simulink model "youBot_Arm"  (R2024a)
settings: Solver=ode15s  StartTime=0.0  StopTime=20  MaxStep=1e-2  RelTol=1e-3  AbsTol=1e-4
model workspace: external: MATLAB File youBot_DataFile.m (data not in the file)
undefined symbols (not defined in the file): Extr_Data_LinkHoles, Qt, sigbuilder_block, smiData, tWP, X, Y, YBT_Par, Z
libraries: sm_lib x193, nesl_utility x130, fl_lib x53, simulink x13, Parts_Lib x10, MyMath_lib x8, Motor_Lib x5, Contact_Forces_Lib x4, ee_lib x2, sdl_lib x2
(part 7 of 8)

== system youBot_Arm/Arm/Environment/Gripper Force/Damper/Gripper Force ==
  Force : Subsystem  mask(Controlled 6-DOF Damping Force){b=contact_b, lpfilt_const_force=lpf_const_gripper_force}
      mask prompts: b "Damping Coefficient"; lpfilt_const_force "Low Pass Filter Constant"
      mask help: Models a controlled 6-DOF damping force. If the distance between two frames is within a certain range (px, py, pz), the damping force is active.
  Measure Apply 6-DOF : sm_lib/Joints/6-DOF Joint  JointMode=Normal  CompositeWrenchDir=FollowerOnBase  CompositeWrenchFrame=BaseFrame  SenseConstraintForce=off  SenseConstraintTorque=off  SenseTotalForce=off  SenseTotalTorque=off  PxPositionTargetSpecify=off  PxPositionTargetPriority=High  PxPositionTargetValue=0  PxPositionTargetValueUnits=m  PxVelocityTargetSpecify=off  PxVelocityTargetPriority=High  PxVelocityTargetValue=0  PxVelocityTargetValueUnits=m/s  PxEquilibriumPosition=0  PxEquilibriumPositionUnits=m  PxSpringStiffness=0  PxSpringStiffnessUnits=N/m  PxDampingCoefficient=0  PxDampingCoefficientUnits=N/(m/s)  PxLowerLimitSpecify=off  PxLowerLimitBound=-1  PxLowerLimitBoundUnits=m  PxLowerLimitStiffness=1e6  PxLowerLimitStiffnessUnits=N/m  PxLowerLimitDamping=1e3  PxLowerLimitDampingUnits=N/(m/s)  PxLowerLimitTransitionRegionWidth=1e-4  PxLowerLimitTransitionRegionWidthUnits=m  PxUpperLimitSpecify=off  PxUpperLimitBound=1  PxUpperLimitBoundUnits=m  PxUpperLimitStiffness=1e6  PxUpperLimitStiffnessUnits=N/m  PxUpperLimitDamping=1e3  PxUpperLimitDampingUnits=N/(m/s)  PxUpperLimitTransitionRegionWidth=1e-4  PxUpperLimitTransitionRegionWidthUnits=m  PxTorqueActuationMode=InputTorque  PxMotionActuationMode=ComputedMotion  PxSensePosition=on  PxSenseVelocity=on  PxSenseAcceleration=off  PxSenseTorqueForce=off  PxSenseLowerLimitTorqueForce=off  PxSenseUpperLimitTorqueForce=off  PyPositionTargetSpecify=off  PyPositionTargetPriority=High  PyPositionTargetValue=40e-2  PyPositionTargetValueUnits=m  PyVelocityTargetSpecify=off  PyVelocityTargetPriority=High  PyVelocityTargetValue=0  PyVelocityTargetValueUnits=m/s  PyEquilibriumPosition=0  PyEquilibriumPositionUnits=m  PySpringStiffness=0  PySpringStiffnessUnits=N/m  PyDampingCoefficient=0  PyDampingCoefficientUnits=N/(m/s)  PyLowerLimitSpecify=off  PyLowerLimitBound=-1  PyLowerLimitBoundUnits=m  PyLowerLimitStiffness=1e6  PyLowerLimitStiffnessUnits=N/m  PyLowerLimitDamping=1e3  PyLowerLimitDampingUnits=N/(m/s)  PyLowerLimitTransitionRegionWidth=1e-4  PyLowerLimitTransitionRegionWidthUnits=m  PyUpperLimitSpecify=off  PyUpperLimitBound=1  PyUpperLimitBoundUnits=m  PyUpperLimitStiffness=1e6  PyUpperLimitStiffnessUnits=N/m  PyUpperLimitDamping=1e3  PyUpperLimitDampingUnits=N/(m/s)  PyUpperLimitTransitionRegionWidth=1e-4  PyUpperLimitTransitionRegionWidthUnits=m  PyTorqueActuationMode=InputTorque  PyMotionActuationMode=ComputedMotion  PySensePosition=on  PySenseVelocity=on  PySenseAcceleration=off  PySenseTorqueForce=off  PySenseLowerLimitTorqueForce=off  PySenseUpperLimitTorqueForce=off  PzPositionTargetSpecify=off  PzPositionTargetPriority=High  PzPositionTargetValue=(YBT_Par.Floor.d+YBT_Par.Cube.d)/2+0.1  PzPositionTargetValueUnits=m  PzVelocityTargetSpecify=off  PzVelocityTargetPriority=High  PzVelocityTargetValue=0  PzVelocityTargetValueUnits=m/s  PzEquilibriumPosition=0  PzEquilibriumPositionUnits=m  PzSpringStiffness=0  PzSpringStiffnessUnits=N/m  PzDampingCoefficient=0  PzDampingCoefficientUnits=N/(m/s)  PzLowerLimitSpecify=off  PzLowerLimitBound=-1  PzLowerLimitBoundUnits=m  PzLowerLimitStiffness=1e6  PzLowerLimitStiffnessUnits=N/m  PzLowerLimitDamping=1e3  PzLowerLimitDampingUnits=N/(m/s)  PzLowerLimitTransitionRegionWidth=1e-4  PzLowerLimitTransitionRegionWidthUnits=m  PzUpperLimitSpecify=off  PzUpperLimitBound=1  PzUpperLimitBoundUnits=m  PzUpperLimitStiffness=1e6  PzUpperLimitStiffnessUnits=N/m  PzUpperLimitDamping=1e3  PzUpperLimitDampingUnits=N/(m/s)  PzUpperLimitTransitionRegionWidth=1e-4  PzUpperLimitTransitionRegionWidthUnits=m  PzTorqueActuationMode=InputTorque  PzMotionActuationMode=ComputedMotion  PzSensePosition=on  PzSenseVelocity=on  PzSenseAcceleration=off  PzSenseTorqueForce=off  PzSenseLowerLimitTorqueForce=off  PzSenseUpperLimitTorqueForce=off  SphPositionTargetSpecify=off  SphPositionTargetPriority=High  SphPositionTargetRotationMethod=None  SphPositionTargetFollAlignAxisA=+X  SphPositionTargetBaseAlignAxisA=+Y  SphPositionTargetFollAlignAxisB=+Y  SphPositionTargetBaseAlignAxisB=+Z  SphPositionTargetRotationStandardAxis=+Z  SphPositionTargetRotationAngle=0.0  SphPositionTargetRotationAngleUnits=deg  SphPositionTargetRotationArbitraryAxis=[0 0 1]  SphPositionTargetRotationSequenceAxes=FollowerAxes  SphPositionTargetRotationSequence=XYX  SphPositionTargetRotationSequenceAngles=[0 0 0]  SphPositionTargetRotationSequenceAnglesUnits=deg  SphPositionTargetRotationMatrix=[1 0 0; 0 1 0; 0 0 1]  SphPositionTargetQuaternion=[1 0 0 0]  SphVelocityTargetSpecify=off  SphVelocityTargetPriority=High  SphVelocityTargetValue=[0 0 0]  SphVelocityTargetValueUnits=deg/s  SphVelocityTargetInFollowerFrame=on  SphEqPosRotationMethod=None  SphEqPosFollAlignAxisA=+X  SphEqPosBaseAlignAxisA=+Y  SphEqPosFollAlignAxisB=+Y  SphEqPosBaseAlignAxisB=+Z  SphEqPosRotationStandardAxis=+Z  SphEqPosRotationAngle=0.0  SphEqPosRotationAngleUnits=deg  SphEqPosRotationArbitraryAxis=[0 0 1]  SphEqPosRotationSequenceAxes=FollowerAxes  SphEqPosRotationSequence=XYX  SphEqPosRotationSequenceAngles=[0 0 0]  SphEqPosRotationSequenceAnglesUnits=deg  SphEqPosRotationMatrix=[1 0 0; 0 1 0; 0 0 1]  SphEqPosQuaternion=[1 0 0 0]  SphSpringStiffness=0  SphSpringStiffnessUnits=N*m/deg  SphDampingCoefficient=0  SphDampingCoefficientUnits=N*m/(deg/s)  SphLowerLimitSpecify=off  SphLowerLimitBound=15  SphLowerLimitBoundUnits=deg  SphLowerLimitStiffness=1e4  SphLowerLimitStiffnessUnits=N*m/deg  SphLowerLimitDamping=10  SphLowerLimitDampingUnits=N*m/(deg/s)  SphLowerLimitTransitionRegionWidth=0.1  SphLowerLimitTransitionRegionWidthUnits=deg  SphUpperLimitSpecify=off  SphUpperLimitBound=45  SphUpperLimitBoundUnits=deg  SphUpperLimitStiffness=1e4  SphUpperLimitStiffnessUnits=N*m/deg  SphUpperLimitDamping=10  SphUpperLimitDampingUnits=N*m/(deg/s)  SphUpperLimitTransitionRegionWidth=0.1  SphUpperLimitTransitionRegionWidthUnits=deg  SphTorqueActuationMode=InputTorque  SphActuateTorqueX=on  SphActuateTorqueY=on  SphActuateTorqueZ=on  SphActuateTorque=off  SphActuationFrame=BaseFrame  SphSensePosition=off  SphSenseVelocityX=on  SphSenseVelocityY=on  SphSenseVelocityZ=on  SphSenseVelocity=off  SphSenseAccelerationX=off  SphSenseAccelerationY=off  SphSenseAccelerationZ=off  SphSenseAcceleration=off  SphSenseLowerLimitTorqueMag=off  SphSenseUpperLimitTorqueMag=off  SphSensingFrame=BaseFrame
  Relative vz : Subsystem  Variant=on  VariantControlMode=label  LabelModeActiveChoice=Housing
      settings: AttributesFormatString=%<ActiveVariant>
  b : PMIOPort  Side=Right
  E : PMIOPort  Port=2  Side=Right
  a : PMIOPort  Port=3  Side=Right
  Box : PMIOPort  Port=4  Side=Left
  connections:
  Force/LConn9 -- Measure Apply 6-DOF/RConn2
  Force/LConn7 -- Measure Apply 6-DOF/RConn4
  Force/LConn5 -- Measure Apply 6-DOF/RConn6
  Force/RConn4 -- Measure Apply 6-DOF/LConn4
  Force/LConn2 -- Measure Apply 6-DOF/RConn9
  Measure Apply 6-DOF/RConn8 -- Force/LConn3
  Force/RConn2 -- Measure Apply 6-DOF/LConn6
  Force/RConn3 -- Measure Apply 6-DOF/LConn5
  Force/RConn6 -- Measure Apply 6-DOF/LConn2
  Measure Apply 6-DOF/LConn3 -- Force/RConn5
  Measure Apply 6-DOF/RConn3 -- Force/LConn8
  Force/LConn6 -- Measure Apply 6-DOF/RConn5
  Force/LConn1 -- Measure Apply 6-DOF/RConn10
  Measure Apply 6-DOF/LConn1 -- a/RConn1
  Measure Apply 6-DOF/RConn1 -- Relative vz/LConn2 -- Box/RConn1
  Measure Apply 6-DOF/LConn7 -- Force/RConn1
  Relative vz/LConn3 -- b/RConn1
  Relative vz/LConn4 -- E/RConn1
  Relative vz/LConn1 -- Measure Apply 6-DOF/RConn7
  Relative vz/RConn1 -- Force/LConn4

== system youBot_Arm/Arm/Environment/Gripper Force/Payload/Marks ==
  Front Rear : sm_lib/Body Elements/Extruded Solid  ExtrusionType=General  PolygonNumSides=3  PolygonOuterRadius=1  PolygonOuterRadiusUnits=m  ExportEntireGeometry=off  ExtrusionCrossSection=YBT_Par.Cube.mark.extrusion  ExtrusionCrossSectionUnits=m  ExportConvexHullGeometry=off  ExtrusionLength=YBT_Par.Cube.d*1.001  ExtrusionLengthUnits=m  InertiaType=PointMass  BasedOnType=Density  Density=1000  DensityUnits=kg/m^3  Mass=0  MassUnits=kg  CenterOfMass=[0 0 0]  CenterOfMassUnits=m  MomentsOfInertia=[1 1 1]  MomentsOfInertiaUnits=kg*m^2  ProductsOfInertia=[1 1 1]  ProductsOfInertiaUnits=kg*m^2  GraphicType=FromGeometry  MarkerShape=Sphere  MarkerSize=10  GraphicVisPropType=SimpleVisualProperties  GraphicDiffuseColor=YBT_Par.Cube.mark.color  GraphicOpacity=1  GraphicSpecularColor=[0.5 0.5 0.5 1.0]  GraphicAmbientColor=[0.15 0.15 0.15 1.0]  GraphicEmissiveColor=[0.0 0.0 0.0 1.0]  GraphicShininess=75  DoExposeReferenceFrame=on  SerializedFrames=<Frames/>
  Left Right : sm_lib/Body Elements/Extruded Solid  ExtrusionType=General  PolygonNumSides=3  PolygonOuterRadius=1  PolygonOuterRadiusUnits=m  ExportEntireGeometry=off  ExtrusionCrossSection=YBT_Par.Cube.mark.extrusion  ExtrusionCrossSectionUnits=m  ExportConvexHullGeometry=off  ExtrusionLength=YBT_Par.Cube.d*1.001  ExtrusionLengthUnits=m  InertiaType=PointMass  BasedOnType=Density  Density=1000  DensityUnits=kg/m^3  Mass=0  MassUnits=kg  CenterOfMass=[0 0 0]  CenterOfMassUnits=m  MomentsOfInertia=[1 1 1]  MomentsOfInertiaUnits=kg*m^2  ProductsOfInertia=[1 1 1]  ProductsOfInertiaUnits=kg*m^2  GraphicType=FromGeometry  MarkerShape=Sphere  MarkerSize=10  GraphicVisPropType=SimpleVisualProperties  GraphicDiffuseColor=YBT_Par.Cube.mark.color  GraphicOpacity=1  GraphicSpecularColor=[0.5 0.5 0.5 1.0]  GraphicAmbientColor=[0.15 0.15 0.15 1.0]  GraphicEmissiveColor=[0.0 0.0 0.0 1.0]  GraphicShininess=75  DoExposeReferenceFrame=on  SerializedFrames=<Frames/>
  Transform Mark Front Rear : sm_lib/Frames and Transforms/Rigid Transform  RotationMethod=StandardAxis  FollAlignAxisA=+X  BaseAlignAxisA=+Y  FollAlignAxisB=+Y  BaseAlignAxisB=+Z  RotationStandardAxis=+X  RotationAngle=90  RotationAngleUnits=deg  RotationArbitraryAxis=[0 0 1]  RotationSequenceAxes=FollowerAxes  RotationSequence=XYX  RotationSequenceAngles=[0 0 0]  RotationSequenceAnglesUnits=deg  RotationMatrix=[1 0 0; 0 1 0; 0 0 1]  Quaternion=[1 0 0 0]  TranslationMethod=None  TranslationCartesianOffset=[0 0 0]  TranslationCartesianOffsetUnits=m  TranslationStandardAxis=+Z  TranslationStandardOffset=0  TranslationStandardOffsetUnits=m  TranslationROffset=0  TranslationROffsetUnits=m  TranslationThetaOffset=0  TranslationThetaOffsetUnits=deg  TranslationZOffset=0  TranslationZOffsetUnits=m
  Transform Mark Left Right : sm_lib/Frames and Transforms/Rigid Transform  RotationMethod=StandardAxis  FollAlignAxisA=+X  BaseAlignAxisA=+Y  FollAlignAxisB=+Y  BaseAlignAxisB=+Z  RotationStandardAxis=+Y  RotationAngle=90  RotationAngleUnits=deg  RotationArbitraryAxis=[0 0 1]  RotationSequenceAxes=FollowerAxes  RotationSequence=XYX  RotationSequenceAngles=[0 0 0]  RotationSequenceAnglesUnits=deg  RotationMatrix=[1 0 0; 0 1 0; 0 0 1]  Quaternion=[1 0 0 0]  TranslationMethod=None  TranslationCartesianOffset=[0 0 0]  TranslationCartesianOffsetUnits=m  TranslationStandardAxis=+Z  TranslationStandardOffset=0  TranslationStandardOffsetUnits=m  TranslationROffset=0  TranslationROffsetUnits=m  TranslationThetaOffset=0  TranslationThetaOffsetUnits=deg  TranslationZOffset=0  TranslationZOffsetUnits=m
  R : PMIOPort  Side=Left
  connections:
  Left Right/RConn1 -- Transform Mark Left Right/RConn1
  Transform Mark Front Rear/RConn1 -- Front Rear/RConn1 -- Transform Mark Left Right/LConn1
  Transform Mark Front Rear/LConn1 -- R/RConn1

== system youBot_Arm/Arm/Environment/Gripper Force/Penalty/Sc2 ==
  In1 : Inport
  Bus Selector1 : BusSelector  OutputSignals=fz1.Normal Force,fz1.Friction Force,fz2.Normal Force,fz2.Friction Force,fz3.Normal Force,fz3.Friction Force,fz4.Normal Force,fz4.Friction Force
  Scope1 : Scope  NumInputPorts=8
  wires:
  Bus Selector1/8 -> Scope1/8  "<Friction Force>"
  Bus Selector1/7 -> Scope1/7  "<Normal Force>"
  Bus Selector1/5 -> Scope1/5  "<Normal Force>"
  In1/1 -> Bus Selector1/1
  Bus Selector1/6 -> Scope1/6  "<Friction Force>"
  Bus Selector1/2 -> Scope1/2  "<Friction Force>"
  Bus Selector1/4 -> Scope1/4  "<Friction Force>"
  Bus Selector1/3 -> Scope1/3  "<Normal Force>"
  Bus Selector1/1 -> Scope1/1  "<Normal Force>"

== system youBot_Arm/Arm/Environment/Load/Box/Camera Frames ==
  Box Left : sm_lib/Frames and Transforms/Rigid Transform  RotationMethod=None  FollAlignAxisA=+X  BaseAlignAxisA=+Y  FollAlignAxisB=+Y  BaseAlignAxisB=+Z  RotationStandardAxis=+Z  RotationAngle=0.0  RotationAngleUnits=deg  RotationArbitraryAxis=[0 0 1]  RotationSequenceAxes=FollowerAxes  RotationSequence=XYX  RotationSequenceAngles=[0 0 0]  RotationSequenceAnglesUnits=deg  RotationMatrix=[1 0 0; 0 1 0; 0 0 1]  Quaternion=[1 0 0 0]  TranslationMethod=StandardAxis  TranslationCartesianOffset=[0 0 0]  TranslationCartesianOffsetUnits=m  TranslationStandardAxis=+X  TranslationStandardOffset=YBT_Par.Cube.d/2+2e-1  TranslationStandardOffsetUnits=m  TranslationROffset=0  TranslationROffsetUnits=m  TranslationThetaOffset=0  TranslationThetaOffsetUnits=deg  TranslationZOffset=0  TranslationZOffsetUnits=m
  Box Rear : sm_lib/Frames and Transforms/Rigid Transform  RotationMethod=None  FollAlignAxisA=+X  BaseAlignAxisA=+Y  FollAlignAxisB=+Y  BaseAlignAxisB=+Z  RotationStandardAxis=+Z  RotationAngle=0.0  RotationAngleUnits=deg  RotationArbitraryAxis=[0 0 1]  RotationSequenceAxes=FollowerAxes  RotationSequence=XYX  RotationSequenceAngles=[0 0 0]  RotationSequenceAnglesUnits=deg  RotationMatrix=[1 0 0; 0 1 0; 0 0 1]  Quaternion=[1 0 0 0]  TranslationMethod=StandardAxis  TranslationCartesianOffset=[0 0 0]  TranslationCartesianOffsetUnits=m  TranslationStandardAxis=+Y  TranslationStandardOffset=YBT_Par.Cube.d/2+2e-1  TranslationStandardOffsetUnits=m  TranslationROffset=0  TranslationROffsetUnits=m  TranslationThetaOffset=0  TranslationThetaOffsetUnits=deg  TranslationZOffset=0  TranslationZOffsetUnits=m
  Box Right : sm_lib/Frames and Transforms/Rigid Transform  RotationMethod=None  FollAlignAxisA=+X  BaseAlignAxisA=+Y  FollAlignAxisB=+Y  BaseAlignAxisB=+Z  RotationStandardAxis=+Z  RotationAngle=0.0  RotationAngleUnits=deg  RotationArbitraryAxis=[0 0 1]  RotationSequenceAxes=FollowerAxes  RotationSequence=XYX  RotationSequenceAngles=[0 0 0]  RotationSequenceAnglesUnits=deg  RotationMatrix=[1 0 0; 0 1 0; 0 0 1]  Quaternion=[1 0 0 0]  TranslationMethod=StandardAxis  TranslationCartesianOffset=[0 0 0]  TranslationCartesianOffsetUnits=m  TranslationStandardAxis=-X  TranslationStandardOffset=YBT_Par.Cube.d/2+2e-1  TranslationStandardOffsetUnits=m  TranslationROffset=0  TranslationROffsetUnits=m  TranslationThetaOffset=0  TranslationThetaOffsetUnits=deg  TranslationZOffset=0  TranslationZOffsetUnits=m
  B : PMIOPort  Side=Left
  connections:
  Box Rear/LConn1 -- Box Left/LConn1 -- Box Right/LConn1 -- B/RConn1

== system youBot_Arm/Arm/Environment/Load/Box/Marks ==
  Front Rear : sm_lib/Body Elements/Extruded Solid  ExtrusionType=General  PolygonNumSides=3  PolygonOuterRadius=1  PolygonOuterRadiusUnits=m  ExportEntireGeometry=off  ExtrusionCrossSection=YBT_Par.Cube.mark.extrusion  ExtrusionCrossSectionUnits=m  ExportConvexHullGeometry=off  ExtrusionLength=YBT_Par.Cube.d*1.001  ExtrusionLengthUnits=m  InertiaType=PointMass  BasedOnType=Density  Density=1000  DensityUnits=kg/m^3  Mass=0  MassUnits=kg  CenterOfMass=[0 0 0]  CenterOfMassUnits=m  MomentsOfInertia=[1 1 1]  MomentsOfInertiaUnits=kg*m^2  ProductsOfInertia=[1 1 1]  ProductsOfInertiaUnits=kg*m^2  GraphicType=FromGeometry  MarkerShape=Sphere  MarkerSize=10  GraphicVisPropType=SimpleVisualProperties  GraphicDiffuseColor=YBT_Par.Cube.mark.color  GraphicOpacity=1.0  GraphicSpecularColor=[0.5 0.5 0.5 1.0]  GraphicAmbientColor=[0.15 0.15 0.15 1.0]  GraphicEmissiveColor=[0.0 0.0 0.0 1.0]  GraphicShininess=75  DoExposeReferenceFrame=on  SerializedFrames=<Frames/>
  Left Right : sm_lib/Body Elements/Extruded Solid  ExtrusionType=General  PolygonNumSides=3  PolygonOuterRadius=1  PolygonOuterRadiusUnits=m  ExportEntireGeometry=off  ExtrusionCrossSection=YBT_Par.Cube.mark.extrusion  ExtrusionCrossSectionUnits=m  ExportConvexHullGeometry=off  ExtrusionLength=YBT_Par.Cube.d*1.001  ExtrusionLengthUnits=m  InertiaType=PointMass  BasedOnType=Density  Density=1000  DensityUnits=kg/m^3  Mass=0  MassUnits=kg  CenterOfMass=[0 0 0]  CenterOfMassUnits=m  MomentsOfInertia=[1 1 1]  MomentsOfInertiaUnits=kg*m^2  ProductsOfInertia=[1 1 1]  ProductsOfInertiaUnits=kg*m^2  GraphicType=FromGeometry  MarkerShape=Sphere  MarkerSize=10  GraphicVisPropType=SimpleVisualProperties  GraphicDiffuseColor=YBT_Par.Cube.mark.color  GraphicOpacity=1.0  GraphicSpecularColor=[0.5 0.5 0.5 1.0]  GraphicAmbientColor=[0.15 0.15 0.15 1.0]  GraphicEmissiveColor=[0.0 0.0 0.0 1.0]  GraphicShininess=75  DoExposeReferenceFrame=on  SerializedFrames=<Frames/>
  Transform Mark Front Rear : sm_lib/Frames and Transforms/Rigid Transform  RotationMethod=StandardAxis  FollAlignAxisA=+X  BaseAlignAxisA=+Y  FollAlignAxisB=+Y  BaseAlignAxisB=+Z  RotationStandardAxis=+X  RotationAngle=90  RotationAngleUnits=deg  RotationArbitraryAxis=[0 0 1]  RotationSequenceAxes=FollowerAxes  RotationSequence=XYX  RotationSequenceAngles=[0 0 0]  RotationSequenceAnglesUnits=deg  RotationMatrix=[1 0 0; 0 1 0; 0 0 1]  Quaternion=[1 0 0 0]  TranslationMethod=None  TranslationCartesianOffset=[0 0 0]  TranslationCartesianOffsetUnits=m  TranslationStandardAxis=+Z  TranslationStandardOffset=0  TranslationStandardOffsetUnits=m  TranslationROffset=0  TranslationROffsetUnits=m  TranslationThetaOffset=0  TranslationThetaOffsetUnits=deg  TranslationZOffset=0  TranslationZOffsetUnits=m
  Transform Mark Left Right : sm_lib/Frames and Transforms/Rigid Transform  RotationMethod=StandardAxis  FollAlignAxisA=+X  BaseAlignAxisA=+Y  FollAlignAxisB=+Y  BaseAlignAxisB=+Z  RotationStandardAxis=+Y  RotationAngle=90  RotationAngleUnits=deg  RotationArbitraryAxis=[0 0 1]  RotationSequenceAxes=FollowerAxes  RotationSequence=XYX  RotationSequenceAngles=[0 0 0]  RotationSequenceAnglesUnits=deg  RotationMatrix=[1 0 0; 0 1 0; 0 0 1]  Quaternion=[1 0 0 0]  TranslationMethod=None  TranslationCartesianOffset=[0 0 0]  TranslationCartesianOffsetUnits=m  TranslationStandardAxis=+Z  TranslationStandardOffset=0  TranslationStandardOffsetUnits=m  TranslationROffset=0  TranslationROffsetUnits=m  TranslationThetaOffset=0  TranslationThetaOffsetUnits=deg  TranslationZOffset=0  TranslationZOffsetUnits=m
  R : PMIOPort  Side=Left
  connections:
  Left Right/RConn1 -- Transform Mark Left Right/RConn1
  Front Rear/RConn1 -- Transform Mark Left Right/LConn1 -- Transform Mark Front Rear/RConn1
  Transform Mark Front Rear/LConn1 -- R/RConn1

== system youBot_Arm/Arm/Actuation/Motor/Bicep/Ideal/Meas B ==
  Bus Creator : BusCreator  Inputs=5
  PS-Simulink Converter : nesl_utility/PS-Simulink Converter  PhysicalDomain=network_engine_domain  SubClassName=ps_output  LeftPortType=input  RightPortType=output  PseudoPeriodic=off  Frequencies=[]  VectorFormat=1-D array  Unit=rad  AffineConversion=off
  PS-Simulink Converter1 : nesl_utility/PS-Simulink Converter  PhysicalDomain=network_engine_domain  SubClassName=ps_output  LeftPortType=input  RightPortType=output  PseudoPeriodic=off  Frequencies=[]  VectorFormat=1-D array  Unit=A  AffineConversion=off
  PS-Simulink Converter2 : nesl_utility/PS-Simulink Converter  PhysicalDomain=network_engine_domain  SubClassName=ps_output  LeftPortType=input  RightPortType=output  PseudoPeriodic=off  Frequencies=[]  VectorFormat=1-D array  Unit=1  AffineConversion=off
  PS-Simulink Converter7 : nesl_utility/PS-Simulink Converter  PhysicalDomain=network_engine_domain  SubClassName=ps_output  LeftPortType=input  RightPortType=output  PseudoPeriodic=off  Frequencies=[]  VectorFormat=1-D array  Unit=rad/s  AffineConversion=off
  PS-Simulink Converter8 : nesl_utility/PS-Simulink Converter  PhysicalDomain=network_engine_domain  SubClassName=ps_output  LeftPortType=input  RightPortType=output  PseudoPeriodic=off  Frequencies=[]  VectorFormat=1-D array  Unit=N*m  AffineConversion=off
  q : PMIOPort  Side=Left
  w : PMIOPort  Port=2  Side=Left
  t : PMIOPort  Port=3  Side=Left
  fc : PMIOPort  Port=4  Side=Left
  i : PMIOPort  Port=5  Side=Left
  B : Outport  VectorParamsAs1DForOutWhenUnconnected=off
  wires:
  Bus Creator/1 -> B/1  "B"
  PS-Simulink Converter8/1 -> Bus Creator/3  "t"
  PS-Simulink Converter7/1 -> Bus Creator/2  "w"
  PS-Simulink Converter/1 -> Bus Creator/1  "q"
  PS-Simulink Converter1/1 -> Bus Creator/4  "i"
  PS-Simulink Converter2/1 -> Bus Creator/5  "fc"
  connections:
  PS-Simulink Converter8/LConn1 -- t/RConn1
  PS-Simulink Converter7/LConn1 -- w/RConn1
  PS-Simulink Converter/LConn1 -- q/RConn1
  PS-Simulink Converter1/LConn1 -- i/RConn1
  PS-Simulink Converter2/LConn1 -- fc/RConn1

== system youBot_Arm/Arm/Actuation/Motor/Bicep/Motor/Meas P ==
  Bus Creator : BusCreator  Inputs=5
  PS-Simulink Converter : nesl_utility/PS-Simulink Converter  PhysicalDomain=network_engine_domain  SubClassName=ps_output  LeftPortType=input  RightPortType=output  PseudoPeriodic=off  Frequencies=[]  VectorFormat=1-D array  Unit=rad  AffineConversion=off
  PS-Simulink Converter1 : nesl_utility/PS-Simulink Converter  PhysicalDomain=network_engine_domain  SubClassName=ps_output  LeftPortType=input  RightPortType=output  PseudoPeriodic=off  Frequencies=[]  VectorFormat=1-D array  Unit=A  AffineConversion=off
  PS-Simulink Converter2 : nesl_utility/PS-Simulink Converter  PhysicalDomain=network_engine_domain  SubClassName=ps_output  LeftPortType=input  RightPortType=output  PseudoPeriodic=off  Frequencies=[]  VectorFormat=1-D array  Unit=1  AffineConversion=off
  PS-Simulink Converter7 : nesl_utility/PS-Simulink Converter  PhysicalDomain=network_engine_domain  SubClassName=ps_output  LeftPortType=input  RightPortType=output  PseudoPeriodic=off  Frequencies=[]  VectorFormat=1-D array  Unit=rad/s  AffineConversion=off
  PS-Simulink Converter8 : nesl_utility/PS-Simulink Converter  PhysicalDomain=network_engine_domain  SubClassName=ps_output  LeftPortType=input  RightPortType=output  PseudoPeriodic=off  Frequencies=[]  VectorFormat=1-D array  Unit=N*m  AffineConversion=off
  q : PMIOPort  Side=Left
  w : PMIOPort  Port=2  Side=Left
  t : PMIOPort  Port=3  Side=Left
  fc : PMIOPort  Port=4  Side=Left
  i : PMIOPort  Port=5  Side=Left
  m : Outport  VectorParamsAs1DForOutWhenUnconnected=off
  wires:
  Bus Creator/1 -> m/1  "B"
  PS-Simulink Converter8/1 -> Bus Creator/3  "t"
  PS-Simulink Converter7/1 -> Bus Creator/2  "w"
  PS-Simulink Converter/1 -> Bus Creator/1  "q"
  PS-Simulink Converter1/1 -> Bus Creator/4  "i"
  PS-Simulink Converter2/1 -> Bus Creator/5  "fc"
  connections:
  PS-Simulink Converter8/LConn1 -- t/RConn1
  PS-Simulink Converter7/LConn1 -- w/RConn1
  PS-Simulink Converter/LConn1 -- q/RConn1
  PS-Simulink Converter1/LConn1 -- i/RConn1
  PS-Simulink Converter2/LConn1 -- fc/RConn1

== system youBot_Arm/Arm/Actuation/Motor/Bicep/Motor/Sensing i ==
  Current Sensor : fl_lib/Electrical/Electrical Sensors/Current Sensor
  i : PMIOPort  Side=Right
  + : PMIOPort  Port=2  Side=Left
  - : PMIOPort  Port=3  Side=Right
  connections:
  Current Sensor/RConn1 -- i/RConn1
  Current Sensor/RConn2 -- -/RConn1
  Current Sensor/LConn1 -- +/RConn1

== system youBot_Arm/Arm/Actuation/Motor/Bicep/Test Motor/Meas P ==
  Bus Creator : BusCreator  Inputs=5
  PS-Simulink Converter : nesl_utility/PS-Simulink Converter  PhysicalDomain=network_engine_domain  SubClassName=ps_output  LeftPortType=input  RightPortType=output  PseudoPeriodic=off  Frequencies=[]  VectorFormat=1-D array  Unit=rad  AffineConversion=off
  PS-Simulink Converter1 : nesl_utility/PS-Simulink Converter  PhysicalDomain=network_engine_domain  SubClassName=ps_output  LeftPortType=input  RightPortType=output  PseudoPeriodic=off  Frequencies=[]  VectorFormat=1-D array  Unit=A  AffineConversion=off
  PS-Simulink Converter2 : nesl_utility/PS-Simulink Converter  PhysicalDomain=network_engine_domain  SubClassName=ps_output  LeftPortType=input  RightPortType=output  PseudoPeriodic=off  Frequencies=[]  VectorFormat=1-D array  Unit=1  AffineConversion=off
  PS-Simulink Converter7 : nesl_utility/PS-Simulink Converter  PhysicalDomain=network_engine_domain  SubClassName=ps_output  LeftPortType=input  RightPortType=output  PseudoPeriodic=off  Frequencies=[]  VectorFormat=1-D array  Unit=rad/s  AffineConversion=off
  PS-Simulink Converter8 : nesl_utility/PS-Simulink Converter  PhysicalDomain=network_engine_domain  SubClassName=ps_output  LeftPortType=input  RightPortType=output  PseudoPeriodic=off  Frequencies=[]  VectorFormat=1-D array  Unit=N*m  AffineConversion=off
  q : PMIOPort  Side=Left
  w : PMIOPort  Port=2  Side=Left
  t : PMIOPort  Port=3  Side=Left
  fc : PMIOPort  Port=4  Side=Left
  i : PMIOPort  Port=5  Side=Left
  P : Outport  VectorParamsAs1DForOutWhenUnconnected=off
  wires:
  Bus Creator/1 -> P/1  "P"
  PS-Simulink Converter8/1 -> Bus Creator/3  "t"
  PS-Simulink Converter7/1 -> Bus Creator/2  "w"
  PS-Simulink Converter/1 -> Bus Creator/1  "q"
  PS-Simulink Converter1/1 -> Bus Creator/4  "i"
  PS-Simulink Converter2/1 -> Bus Creator/5  "fc"
  connections:
  PS-Simulink Converter8/LConn1 -- t/RConn1
  PS-Simulink Converter7/LConn1 -- w/RConn1
  PS-Simulink Converter/LConn1 -- q/RConn1
  PS-Simulink Converter1/LConn1 -- i/RConn1
  PS-Simulink Converter2/LConn1 -- fc/RConn1

== system youBot_Arm/Arm/Actuation/Motor/Forearm/Ideal/Meas F ==
  Bus Creator : BusCreator  Inputs=5
  PS-Simulink Converter : nesl_utility/PS-Simulink Converter  PhysicalDomain=network_engine_domain  SubClassName=ps_output  LeftPortType=input  RightPortType=output  PseudoPeriodic=off  Frequencies=[]  VectorFormat=1-D array  Unit=rad  AffineConversion=off
  PS-Simulink Converter1 : nesl_utility/PS-Simulink Converter  PhysicalDomain=network_engine_domain  SubClassName=ps_output  LeftPortType=input  RightPortType=output  PseudoPeriodic=off  Frequencies=[]  VectorFormat=1-D array  Unit=A  AffineConversion=off
  PS-Simulink Converter2 : nesl_utility/PS-Simulink Converter  PhysicalDomain=network_engine_domain  SubClassName=ps_output  LeftPortType=input  RightPortType=output  PseudoPeriodic=off  Frequencies=[]  VectorFormat=1-D array  Unit=1  AffineConversion=off
  PS-Simulink Converter7 : nesl_utility/PS-Simulink Converter  PhysicalDomain=network_engine_domain  SubClassName=ps_output  LeftPortType=input  RightPortType=output  PseudoPeriodic=off  Frequencies=[]  VectorFormat=1-D array  Unit=rad/s  AffineConversion=off
  PS-Simulink Converter8 : nesl_utility/PS-Simulink Converter  PhysicalDomain=network_engine_domain  SubClassName=ps_output  LeftPortType=input  RightPortType=output  PseudoPeriodic=off  Frequencies=[]  VectorFormat=1-D array  Unit=N*m  AffineConversion=off
  q : PMIOPort  Side=Left
  w : PMIOPort  Port=2  Side=Left
  t : PMIOPort  Port=3  Side=Left
  fc : PMIOPort  Port=4  Side=Left
  i : PMIOPort  Port=5  Side=Left
  F : Outport  VectorParamsAs1DForOutWhenUnconnected=off
  wires:
  PS-Simulink Converter/1 -> Bus Creator/1  "q"
  PS-Simulink Converter7/1 -> Bus Creator/2  "w"
  PS-Simulink Converter8/1 -> Bus Creator/3  "t"
  Bus Creator/1 -> F/1  "F"
  PS-Simulink Converter1/1 -> Bus Creator/4  "i"
  PS-Simulink Converter2/1 -> Bus Creator/5  "fc"
  connections:
  PS-Simulink Converter/LConn1 -- q/RConn1
  PS-Simulink Converter7/LConn1 -- w/RConn1
  PS-Simulink Converter8/LConn1 -- t/RConn1
  PS-Simulink Converter1/LConn1 -- i/RConn1
  PS-Simulink Converter2/LConn1 -- fc/RConn1

== system youBot_Arm/Arm/Actuation/Motor/Forearm/Motor/Meas P ==
  Bus Creator : BusCreator  Inputs=5
  PS-Simulink Converter : nesl_utility/PS-Simulink Converter  PhysicalDomain=network_engine_domain  SubClassName=ps_output  LeftPortType=input  RightPortType=output  PseudoPeriodic=off  Frequencies=[]  VectorFormat=1-D array  Unit=rad  AffineConversion=off
  PS-Simulink Converter1 : nesl_utility/PS-Simulink Converter  PhysicalDomain=network_engine_domain  SubClassName=ps_output  LeftPortType=input  RightPortType=output  PseudoPeriodic=off  Frequencies=[]  VectorFormat=1-D array  Unit=A  AffineConversion=off
  PS-Simulink Converter2 : nesl_utility/PS-Simulink Converter  PhysicalDomain=network_engine_domain  SubClassName=ps_output  LeftPortType=input  RightPortType=output  PseudoPeriodic=off  Frequencies=[]  VectorFormat=1-D array  Unit=1  AffineConversion=off
  PS-Simulink Converter7 : nesl_utility/PS-Simulink Converter  PhysicalDomain=network_engine_domain  SubClassName=ps_output  LeftPortType=input  RightPortType=output  PseudoPeriodic=off  Frequencies=[]  VectorFormat=1-D array  Unit=rad/s  AffineConversion=off
  PS-Simulink Converter8 : nesl_utility/PS-Simulink Converter  PhysicalDomain=network_engine_domain  SubClassName=ps_output  LeftPortType=input  RightPortType=output  PseudoPeriodic=off  Frequencies=[]  VectorFormat=1-D array  Unit=N*m  AffineConversion=off
  q : PMIOPort  Side=Left
  w : PMIOPort  Port=2  Side=Left
  t : PMIOPort  Port=3  Side=Left
  fc : PMIOPort  Port=4  Side=Left
  i : PMIOPort  Port=5  Side=Left
  m : Outport  VectorParamsAs1DForOutWhenUnconnected=off
  wires:
  Bus Creator/1 -> m/1  "F"
  PS-Simulink Converter8/1 -> Bus Creator/3  "t"
  PS-Simulink Converter7/1 -> Bus Creator/2  "w"
  PS-Simulink Converter/1 -> Bus Creator/1  "q"
  PS-Simulink Converter1/1 -> Bus Creator/4  "i"
  PS-Simulink Converter2/1 -> Bus Creator/5  "fc"
  connections:
  PS-Simulink Converter8/LConn1 -- t/RConn1
  PS-Simulink Converter7/LConn1 -- w/RConn1
  PS-Simulink Converter/LConn1 -- q/RConn1
  PS-Simulink Converter1/LConn1 -- i/RConn1
  PS-Simulink Converter2/LConn1 -- fc/RConn1

== system youBot_Arm/Arm/Actuation/Motor/Forearm/Motor/Sensing i ==
  Current Sensor : fl_lib/Electrical/Electrical Sensors/Current Sensor
  i : PMIOPort  Side=Right
  + : PMIOPort  Port=2  Side=Left
  - : PMIOPort  Port=3  Side=Right
  connections:
  Current Sensor/RConn1 -- i/RConn1
  Current Sensor/RConn2 -- -/RConn1
  Current Sensor/LConn1 -- +/RConn1

== system youBot_Arm/Arm/Actuation/Motor/Gripper/Ideal/Meas G ==
  Bus Creator : BusCreator  Inputs=5
  PS-Simulink Converter : nesl_utility/PS-Simulink Converter  PhysicalDomain=network_engine_domain  SubClassName=ps_output  LeftPortType=input  RightPortType=output  PseudoPeriodic=off  Frequencies=[]  VectorFormat=1-D array  Unit=rad  AffineConversion=off
  PS-Simulink Converter1 : nesl_utility/PS-Simulink Converter  PhysicalDomain=network_engine_domain  SubClassName=ps_output  LeftPortType=input  RightPortType=output  PseudoPeriodic=off  Frequencies=[]  VectorFormat=1-D array  Unit=A  AffineConversion=off
  PS-Simulink Converter2 : nesl_utility/PS-Simulink Converter  PhysicalDomain=network_engine_domain  SubClassName=ps_output  LeftPortType=input  RightPortType=output  PseudoPeriodic=off  Frequencies=[]  VectorFormat=1-D array  Unit=1  AffineConversion=off
  PS-Simulink Converter7 : nesl_utility/PS-Simulink Converter  PhysicalDomain=network_engine_domain  SubClassName=ps_output  LeftPortType=input  RightPortType=output  PseudoPeriodic=off  Frequencies=[]  VectorFormat=1-D array  Unit=rad/s  AffineConversion=off
  PS-Simulink Converter8 : nesl_utility/PS-Simulink Converter  PhysicalDomain=network_engine_domain  SubClassName=ps_output  LeftPortType=input  RightPortType=output  PseudoPeriodic=off  Frequencies=[]  VectorFormat=1-D array  Unit=N*m  AffineConversion=off
  q : PMIOPort  Side=Left
  w : PMIOPort  Port=2  Side=Left
  t : PMIOPort  Port=3  Side=Left
  fc : PMIOPort  Port=4  Side=Left
  i : PMIOPort  Port=5  Side=Left
  G : Outport  VectorParamsAs1DForOutWhenUnconnected=off
  wires:
  Bus Creator/1 -> G/1  "G"
  PS-Simulink Converter8/1 -> Bus Creator/3  "t"
  PS-Simulink Converter7/1 -> Bus Creator/2  "w"
  PS-Simulink Converter/1 -> Bus Creator/1  "q"
  PS-Simulink Converter1/1 -> Bus Creator/4  "i"
  PS-Simulink Converter2/1 -> Bus Creator/5  "fc"
  connections:
  PS-Simulink Converter8/LConn1 -- t/RConn1
  PS-Simulink Converter7/LConn1 -- w/RConn1
  PS-Simulink Converter/LConn1 -- q/RConn1
  PS-Simulink Converter1/LConn1 -- i/RConn1
  PS-Simulink Converter2/LConn1 -- fc/RConn1

== system youBot_Arm/Arm/Actuation/Motor/Gripper/Motor/Meas P ==
  Bus Creator : BusCreator  Inputs=5
  PS-Simulink Converter : nesl_utility/PS-Simulink Converter  PhysicalDomain=network_engine_domain  SubClassName=ps_output  LeftPortType=input  RightPortType=output  PseudoPeriodic=off  Frequencies=[]  VectorFormat=1-D array  Unit=rad  AffineConversion=off
  PS-Simulink Converter1 : nesl_utility/PS-Simulink Converter  PhysicalDomain=network_engine_domain  SubClassName=ps_output  LeftPortType=input  RightPortType=output  PseudoPeriodic=off  Frequencies=[]  VectorFormat=1-D array  Unit=A  AffineConversion=off
  PS-Simulink Converter2 : nesl_utility/PS-Simulink Converter  PhysicalDomain=network_engine_domain  SubClassName=ps_output  LeftPortType=input  RightPortType=output  PseudoPeriodic=off  Frequencies=[]  VectorFormat=1-D array  Unit=1  AffineConversion=off
  PS-Simulink Converter7 : nesl_utility/PS-Simulink Converter  PhysicalDomain=network_engine_domain  SubClassName=ps_output  LeftPortType=input  RightPortType=output  PseudoPeriodic=off  Frequencies=[]  VectorFormat=1-D array  Unit=rad/s  AffineConversion=off
  PS-Simulink Converter8 : nesl_utility/PS-Simulink Converter  PhysicalDomain=network_engine_domain  SubClassName=ps_output  LeftPortType=input  RightPortType=output  PseudoPeriodic=off  Frequencies=[]  VectorFormat=1-D array  Unit=N*m  AffineConversion=off
  q : PMIOPort  Side=Left
  w : PMIOPort  Port=2  Side=Left
  t : PMIOPort  Port=3  Side=Left
  fc : PMIOPort  Port=4  Side=Left
  i : PMIOPort  Port=5  Side=Left
  m : Outport  VectorParamsAs1DForOutWhenUnconnected=off
  wires:
  Bus Creator/1 -> m/1  "G"
  PS-Simulink Converter8/1 -> Bus Creator/3  "t"
  PS-Simulink Converter7/1 -> Bus Creator/2  "w"
  PS-Simulink Converter/1 -> Bus Creator/1  "q"
  PS-Simulink Converter1/1 -> Bus Creator/4  "i"
  PS-Simulink Converter2/1 -> Bus Creator/5  "fc"
  connections:
  PS-Simulink Converter8/LConn1 -- t/RConn1
  PS-Simulink Converter7/LConn1 -- w/RConn1
  PS-Simulink Converter/LConn1 -- q/RConn1
  PS-Simulink Converter1/LConn1 -- i/RConn1
  PS-Simulink Converter2/LConn1 -- fc/RConn1

== system youBot_Arm/Arm/Actuation/Motor/Gripper/Motor/Sensing i ==
  Current Sensor : fl_lib/Electrical/Electrical Sensors/Current Sensor
  i : PMIOPort  Side=Right
  + : PMIOPort  Port=2  Side=Left
  - : PMIOPort  Port=3  Side=Right
  connections:
  Current Sensor/RConn1 -- i/RConn1
  Current Sensor/RConn2 -- -/RConn1
  Current Sensor/LConn1 -- +/RConn1

== system youBot_Arm/Arm/Actuation/Motor/Pivot/Ideal/Meas P ==
  Bus Creator : BusCreator  Inputs=5
  PS-Simulink Converter : nesl_utility/PS-Simulink Converter  PhysicalDomain=network_engine_domain  SubClassName=ps_output  LeftPortType=input  RightPortType=output  PseudoPeriodic=off  Frequencies=[]  VectorFormat=1-D array  Unit=rad  AffineConversion=off
  PS-Simulink Converter1 : nesl_utility/PS-Simulink Converter  PhysicalDomain=network_engine_domain  SubClassName=ps_output  LeftPortType=input  RightPortType=output  PseudoPeriodic=off  Frequencies=[]  VectorFormat=1-D array  Unit=A  AffineConversion=off
  PS-Simulink Converter2 : nesl_utility/PS-Simulink Converter  PhysicalDomain=network_engine_domain  SubClassName=ps_output  LeftPortType=input  RightPortType=output  PseudoPeriodic=off  Frequencies=[]  VectorFormat=1-D array  Unit=1  AffineConversion=off
  PS-Simulink Converter7 : nesl_utility/PS-Simulink Converter  PhysicalDomain=network_engine_domain  SubClassName=ps_output  LeftPortType=input  RightPortType=output  PseudoPeriodic=off  Frequencies=[]  VectorFormat=1-D array  Unit=rad/s  AffineConversion=off
  PS-Simulink Converter8 : nesl_utility/PS-Simulink Converter  PhysicalDomain=network_engine_domain  SubClassName=ps_output  LeftPortType=input  RightPortType=output  PseudoPeriodic=off  Frequencies=[]  VectorFormat=1-D array  Unit=N*m  AffineConversion=off
  q : PMIOPort  Side=Left
  w : PMIOPort  Port=2  Side=Left
  t : PMIOPort  Port=3  Side=Left
  fc : PMIOPort  Port=4  Side=Left
  i : PMIOPort  Port=5  Side=Left
  P : Outport  VectorParamsAs1DForOutWhenUnconnected=off
  wires:
  Bus Creator/1 -> P/1  "P"
  PS-Simulink Converter8/1 -> Bus Creator/3  "t"
  PS-Simulink Converter7/1 -> Bus Creator/2  "w"
  PS-Simulink Converter/1 -> Bus Creator/1  "q"
  PS-Simulink Converter1/1 -> Bus Creator/4  "i"
  PS-Simulink Converter2/1 -> Bus Creator/5  "fc"
  connections:
  PS-Simulink Converter8/LConn1 -- t/RConn1
  PS-Simulink Converter7/LConn1 -- w/RConn1
  PS-Simulink Converter/LConn1 -- q/RConn1
  PS-Simulink Converter1/LConn1 -- i/RConn1
  PS-Simulink Converter2/LConn1 -- fc/RConn1

== system youBot_Arm/Arm/Actuation/Motor/Pivot/Motor/Meas P ==
  Bus Creator : BusCreator  Inputs=5
  PS-Simulink Converter : nesl_utility/PS-Simulink Converter  PhysicalDomain=network_engine_domain  SubClassName=ps_output  LeftPortType=input  RightPortType=output  PseudoPeriodic=off  Frequencies=[]  VectorFormat=1-D array  Unit=rad  AffineConversion=off
  PS-Simulink Converter1 : nesl_utility/PS-Simulink Converter  PhysicalDomain=network_engine_domain  SubClassName=ps_output  LeftPortType=input  RightPortType=output  PseudoPeriodic=off  Frequencies=[]  VectorFormat=1-D array  Unit=A  AffineConversion=off
  PS-Simulink Converter2 : nesl_utility/PS-Simulink Converter  PhysicalDomain=network_engine_domain  SubClassName=ps_output  LeftPortType=input  RightPortType=output  PseudoPeriodic=off  Frequencies=[]  VectorFormat=1-D array  Unit=1  AffineConversion=off
  PS-Simulink Converter7 : nesl_utility/PS-Simulink Converter  PhysicalDomain=network_engine_domain  SubClassName=ps_output  LeftPortType=input  RightPortType=output  PseudoPeriodic=off  Frequencies=[]  VectorFormat=1-D array  Unit=rad/s  AffineConversion=off
  PS-Simulink Converter8 : nesl_utility/PS-Simulink Converter  PhysicalDomain=network_engine_domain  SubClassName=ps_output  LeftPortType=input  RightPortType=output  PseudoPeriodic=off  Frequencies=[]  VectorFormat=1-D array  Unit=N*m  AffineConversion=off
  q : PMIOPort  Side=Left
  w : PMIOPort  Port=2  Side=Left
  t : PMIOPort  Port=3  Side=Left
  fc : PMIOPort  Port=4  Side=Left
  i : PMIOPort  Port=5  Side=Left
  P : Outport  VectorParamsAs1DForOutWhenUnconnected=off
  wires:
  Bus Creator/1 -> P/1  "P"
  PS-Simulink Converter8/1 -> Bus Creator/3  "t"
  PS-Simulink Converter7/1 -> Bus Creator/2  "w"
  PS-Simulink Converter/1 -> Bus Creator/1  "q"
  PS-Simulink Converter1/1 -> Bus Creator/4  "i"
  PS-Simulink Converter2/1 -> Bus Creator/5  "fc"
  connections:
  PS-Simulink Converter8/LConn1 -- t/RConn1
  PS-Simulink Converter7/LConn1 -- w/RConn1
  PS-Simulink Converter/LConn1 -- q/RConn1
  PS-Simulink Converter1/LConn1 -- i/RConn1
  PS-Simulink Converter2/LConn1 -- fc/RConn1

== system youBot_Arm/Arm/Actuation/Motor/Pivot/Motor/Sensing i ==
  Current Sensor : fl_lib/Electrical/Electrical Sensors/Current Sensor
  i : PMIOPort  Side=Right
  + : PMIOPort  Port=2  Side=Left
  - : PMIOPort  Port=3  Side=Right
  connections:
  Current Sensor/RConn1 -- i/RConn1
  Current Sensor/RConn2 -- -/RConn1
  Current Sensor/LConn1 -- +/RConn1

== system youBot_Arm/Arm/Actuation/Motor/Pivot/Test Motor/Meas P ==
  Bus Creator : BusCreator  Inputs=5
  PS-Simulink Converter : nesl_utility/PS-Simulink Converter  PhysicalDomain=network_engine_domain  SubClassName=ps_output  LeftPortType=input  RightPortType=output  PseudoPeriodic=off  Frequencies=[]  VectorFormat=1-D array  Unit=rad  AffineConversion=off
  PS-Simulink Converter1 : nesl_utility/PS-Simulink Converter  PhysicalDomain=network_engine_domain  SubClassName=ps_output  LeftPortType=input  RightPortType=output  PseudoPeriodic=off  Frequencies=[]  VectorFormat=1-D array  Unit=A  AffineConversion=off
  PS-Simulink Converter2 : nesl_utility/PS-Simulink Converter  PhysicalDomain=network_engine_domain  SubClassName=ps_output  LeftPortType=input  RightPortType=output  PseudoPeriodic=off  Frequencies=[]  VectorFormat=1-D array  Unit=1  AffineConversion=off
  PS-Simulink Converter7 : nesl_utility/PS-Simulink Converter  PhysicalDomain=network_engine_domain  SubClassName=ps_output  LeftPortType=input  RightPortType=output  PseudoPeriodic=off  Frequencies=[]  VectorFormat=1-D array  Unit=rad/s  AffineConversion=off
  PS-Simulink Converter8 : nesl_utility/PS-Simulink Converter  PhysicalDomain=network_engine_domain  SubClassName=ps_output  LeftPortType=input  RightPortType=output  PseudoPeriodic=off  Frequencies=[]  VectorFormat=1-D array  Unit=N*m  AffineConversion=off
  q : PMIOPort  Side=Left
  w : PMIOPort  Port=2  Side=Left
  t : PMIOPort  Port=3  Side=Left
  fc : PMIOPort  Port=4  Side=Left
  i : PMIOPort  Port=5  Side=Left
  P : Outport  VectorParamsAs1DForOutWhenUnconnected=off
  wires:
  Bus Creator/1 -> P/1  "P"
  PS-Simulink Converter8/1 -> Bus Creator/3  "t"
  PS-Simulink Converter7/1 -> Bus Creator/2  "w"
  PS-Simulink Converter/1 -> Bus Creator/1  "q"
  PS-Simulink Converter1/1 -> Bus Creator/4  "i"
  PS-Simulink Converter2/1 -> Bus Creator/5  "fc"
  connections:
  PS-Simulink Converter8/LConn1 -- t/RConn1
  PS-Simulink Converter7/LConn1 -- w/RConn1
  PS-Simulink Converter/LConn1 -- q/RConn1
  PS-Simulink Converter1/LConn1 -- i/RConn1
  PS-Simulink Converter2/LConn1 -- fc/RConn1

== system youBot_Arm/Arm/Actuation/Motor/Wrist/Ideal/Meas W ==
  Bus Creator : BusCreator  Inputs=5
  PS-Simulink Converter : nesl_utility/PS-Simulink Converter  PhysicalDomain=network_engine_domain  SubClassName=ps_output  LeftPortType=input  RightPortType=output  PseudoPeriodic=off  Frequencies=[]  VectorFormat=1-D array  Unit=rad  AffineConversion=off
  PS-Simulink Converter1 : nesl_utility/PS-Simulink Converter  PhysicalDomain=network_engine_domain  SubClassName=ps_output  LeftPortType=input  RightPortType=output  PseudoPeriodic=off  Frequencies=[]  VectorFormat=1-D array  Unit=A  AffineConversion=off
  PS-Simulink Converter2 : nesl_utility/PS-Simulink Converter  PhysicalDomain=network_engine_domain  SubClassName=ps_output  LeftPortType=input  RightPortType=output  PseudoPeriodic=off  Frequencies=[]  VectorFormat=1-D array  Unit=1  AffineConversion=off
  PS-Simulink Converter7 : nesl_utility/PS-Simulink Converter  PhysicalDomain=network_engine_domain  SubClassName=ps_output  LeftPortType=input  RightPortType=output  PseudoPeriodic=off  Frequencies=[]  VectorFormat=1-D array  Unit=rad/s  AffineConversion=off
  PS-Simulink Converter8 : nesl_utility/PS-Simulink Converter  PhysicalDomain=network_engine_domain  SubClassName=ps_output  LeftPortType=input  RightPortType=output  PseudoPeriodic=off  Frequencies=[]  VectorFormat=1-D array  Unit=N*m  AffineConversion=off
  q : PMIOPort  Side=Left
  w : PMIOPort  Port=2  Side=Left
  t : PMIOPort  Port=3  Side=Left
  fc : PMIOPort  Port=4  Side=Left
  i : PMIOPort  Port=5  Side=Left
  W : Outport  VectorParamsAs1DForOutWhenUnconnected=off
  wires:
  PS-Simulink Converter/1 -> Bus Creator/1  "q"
  PS-Simulink Converter7/1 -> Bus Creator/2  "w"
  PS-Simulink Converter8/1 -> Bus Creator/3  "t"
  Bus Creator/1 -> W/1  "W"
  PS-Simulink Converter1/1 -> Bus Creator/4  "i"
  PS-Simulink Converter2/1 -> Bus Creator/5  "fc"
  connections:
  PS-Simulink Converter/LConn1 -- q/RConn1
  PS-Simulink Converter7/LConn1 -- w/RConn1
  PS-Simulink Converter8/LConn1 -- t/RConn1
  PS-Simulink Converter1/LConn1 -- i/RConn1
  PS-Simulink Converter2/LConn1 -- fc/RConn1

== system youBot_Arm/Arm/Actuation/Motor/Wrist/Motor/Meas P ==
  Bus Creator : BusCreator  Inputs=5
  PS-Simulink Converter : nesl_utility/PS-Simulink Converter  PhysicalDomain=network_engine_domain  SubClassName=ps_output  LeftPortType=input  RightPortType=output  PseudoPeriodic=off  Frequencies=[]  VectorFormat=1-D array  Unit=rad  AffineConversion=off
  PS-Simulink Converter1 : nesl_utility/PS-Simulink Converter  PhysicalDomain=network_engine_domain  SubClassName=ps_output  LeftPortType=input  RightPortType=output  PseudoPeriodic=off  Frequencies=[]  VectorFormat=1-D array  Unit=A  AffineConversion=off
  PS-Simulink Converter2 : nesl_utility/PS-Simulink Converter  PhysicalDomain=network_engine_domain  SubClassName=ps_output  LeftPortType=input  RightPortType=output  PseudoPeriodic=off  Frequencies=[]  VectorFormat=1-D array  Unit=1  AffineConversion=off
  PS-Simulink Converter7 : nesl_utility/PS-Simulink Converter  PhysicalDomain=network_engine_domain  SubClassName=ps_output  LeftPortType=input  RightPortType=output  PseudoPeriodic=off  Frequencies=[]  VectorFormat=1-D array  Unit=rad/s  AffineConversion=off
  PS-Simulink Converter8 : nesl_utility/PS-Simulink Converter  PhysicalDomain=network_engine_domain  SubClassName=ps_output  LeftPortType=input  RightPortType=output  PseudoPeriodic=off  Frequencies=[]  VectorFormat=1-D array  Unit=N*m  AffineConversion=off
  q : PMIOPort  Side=Left
  w : PMIOPort  Port=2  Side=Left
  t : PMIOPort  Port=3  Side=Left
  fc : PMIOPort  Port=4  Side=Left
  i : PMIOPort  Port=5  Side=Left
  m : Outport  VectorParamsAs1DForOutWhenUnconnected=off
  wires:
  Bus Creator/1 -> m/1  "W"
  PS-Simulink Converter8/1 -> Bus Creator/3  "t"
  PS-Simulink Converter7/1 -> Bus Creator/2  "w"
  PS-Simulink Converter/1 -> Bus Creator/1  "q"
  PS-Simulink Converter1/1 -> Bus Creator/4  "i"
  PS-Simulink Converter2/1 -> Bus Creator/5  "fc"
  connections:
  PS-Simulink Converter8/LConn1 -- t/RConn1
  PS-Simulink Converter7/LConn1 -- w/RConn1
  PS-Simulink Converter/LConn1 -- q/RConn1
  PS-Simulink Converter1/LConn1 -- i/RConn1
  PS-Simulink Converter2/LConn1 -- fc/RConn1

== system youBot_Arm/Arm/Actuation/Motor/Wrist/Motor/Sensing i ==
  Current Sensor : fl_lib/Electrical/Electrical Sensors/Current Sensor
  i : PMIOPort  Side=Right
  + : PMIOPort  Port=2  Side=Left
  - : PMIOPort  Port=3  Side=Right
  connections:
  Current Sensor/RConn1 -- i/RConn1
  Current Sensor/RConn2 -- -/RConn1
  Current Sensor/LConn1 -- +/RConn1
